simulink model "RCC_OCC_TS_TYPE1_HL"  (Simulink 7.7)
settings: Solver=ode1  StartTime=0.0  StopTime=inf  FixedStep=2e-5  RelTol=1e-3
libraries: powerlib x28, rtio_opalrt_common x4, rtlab x2
settings Model: Creator=bbkon  LastModifiedBy=USER
settings SolverCC: AutoInsertRateTranBlk=on

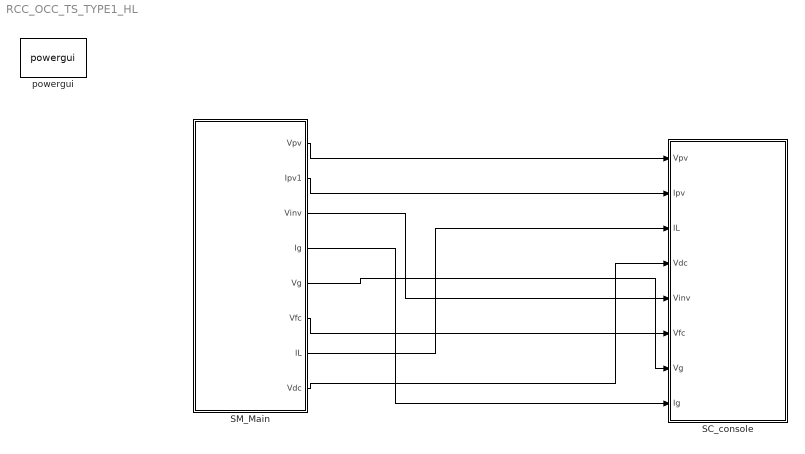
== system RCC_OCC_TS_TYPE1_HL ==
  SC_console : Subsystem
  SM_Main : Subsystem
  powergui : powerlib/powergui  Priority=1  SystemSampleTime=-1  SimulationMode=Discrete  SampleTime=2e-5  frequency=60  SPID=off  DisableSnubberDevices=off  DisableRonSwitches=off  DisableVfSwitches=off  SwTol=0  Interpol=off  DisplayEquations=off  FunctionMessages=off  frequencyindice=0  Pbase=100e6  ErrMax=1e-4  Iterations=50  UnitsV=kV  UnitsW=MW  echomessages=off  HookPort=off  EnableUseOfTLC=off  x0status=blocks  RestoreLinks=warning  ResistiveCurrentMeasurement=off  Ylog=off  Xlog=on  ShowGrid=off  save=off  variable=ZData  ZoomFFT=off  StartTime=0.0  cycles=1  DisplayStyle=1  FreqAxis=off  MaxFrequency=1000  frequencyindicesteady=1  display=off  methode=off
  wires:
  SM_Main/1(Vpv) -> SC_console/1(Vpv)
  SM_Main/2(Ipv1) -> SC_console/2(Ipv)
  SM_Main/3(Vinv) -> SC_console/5(Vinv)
  SM_Main/4(Ig) -> SC_console/8(Ig)
  SM_Main/5(Vg) -> SC_console/7(Vg)
  SM_Main/6(Vfc) -> SC_console/6(Vfc)
  SM_Main/7(IL) -> SC_console/3(IL)
  SM_Main/8(Vdc) -> SC_console/4(Vdc)

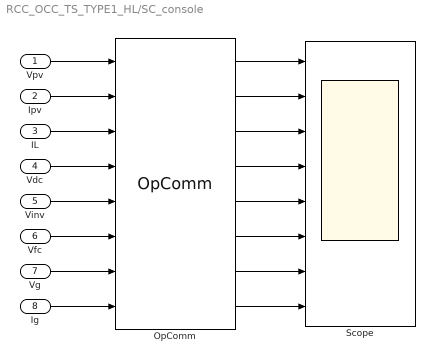
== system RCC_OCC_TS_TYPE1_HL/SC_console ==
  Vpv : Inport
  Ipv : Inport  Port=2
  IL : Inport  Port=3
  Vdc : Inport  Port=4
  Vinv : Inport  Port=5
  Vfc : Inport  Port=6
  Vg : Inport  Port=7
  Ig : Inport  Port=8
  OpComm : rtlab/OpComm  SystemSampleTime=-1  nbport=8  groupe_acq=1  subsys_rate=0  st=0  Synchronization=on  Interpolation=on  Threshold=1.0  Missed_Data=off  Sim_Time=off  Samples=off  dynSigOut=off  from_console=0  warning_done=off  writeOpCommFile=off  Offset=off
  Scope : Scope  NumInputPorts=8
      settings: YMin=80~7.25~6.5~394~-500~399~-400~-7.5  YMax=125~9.75~11.5~405~500~408~400~7.5
  wires:
  Vpv/1 -> OpComm/1
  Ipv/1 -> OpComm/2
  IL/1 -> OpComm/3
  Vdc/1 -> OpComm/4
  Vinv/1 -> OpComm/5
  Vfc/1 -> OpComm/6
  Vg/1 -> OpComm/7
  Ig/1 -> OpComm/8
  OpComm/1 -> Scope/1
  OpComm/2 -> Scope/2
  OpComm/3 -> Scope/3
  OpComm/4 -> Scope/4
  OpComm/5 -> Scope/5
  OpComm/6 -> Scope/6
  OpComm/7 -> Scope/7
  OpComm/8 -> Scope/8

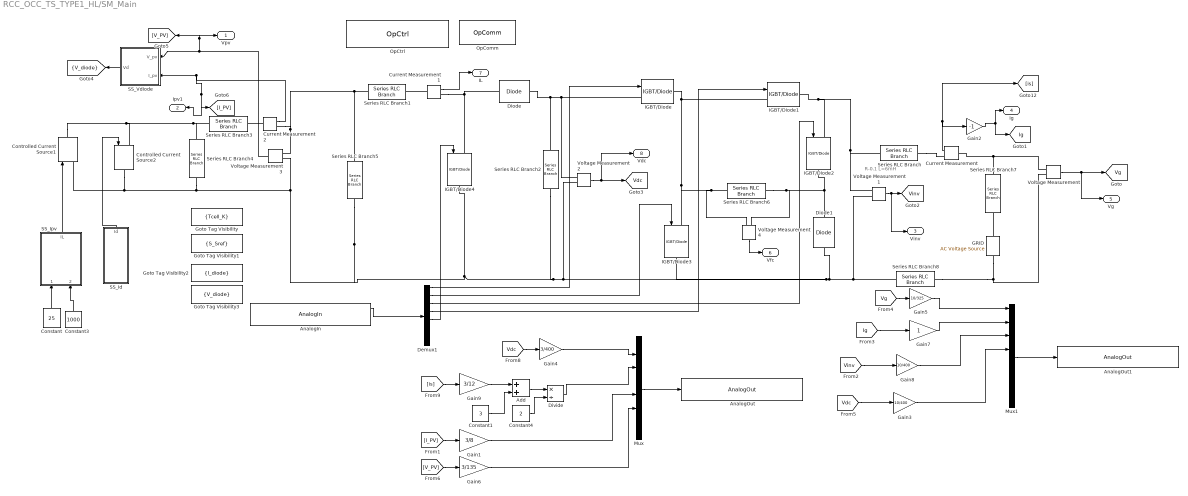
== system RCC_OCC_TS_TYPE1_HL/SM_Main ==
  note: R-0.1 L=6mH
  Add : Sum
  AnalogIn : rtio_opalrt_common/AnalogIn  CtrlName='OpCtrl'  portNb=1  FcnNos=Slot 2 Module A Subsection 1  size=16  maxcount=8  count=8  numchan=8  sampleTime=2e-5
      settings: AttributesFormatString=%<CtrlName>
  AnalogOut : rtio_opalrt_common/AnalogOut  CtrlName='OpCtrl'  portNb=1  FcnNos=Slot 2 Module B Subsection 1  size=16  maxcount=8  count=8  numchan=8  israngeinput=off  voltagerange=[-16 ... 16]  slot=1  side=1  mismatch=0  slotside=Slot_2_Module_B
      settings: AttributesFormatString=%<CtrlName>
  AnalogOut1 : rtio_opalrt_common/AnalogOut  CtrlName='OpCtrl'  portNb=2  FcnNos=Slot 2 Module B Subsection 2  size=16  maxcount=8  count=8  numchan=8  israngeinput=off  voltagerange=[-16 ... 16]  slot=1  side=1  mismatch=0  slotside=Slot_2_Module_B
      settings: AttributesFormatString=%<CtrlName>
  Constant : Constant  Value=25
  Constant1 : Constant  Value=3  SampleTime=-1
  Constant3 : Constant  Value=1000
  Constant4 : Constant  Value=2  SampleTime=-1
  Controlled Current Source1 : powerlib/Electrical Sources/Controlled Current Source  SystemSampleTime=-1  Initialize=on  Source_Type=AC  Amplitude=0  Phase=0  Frequency=0  Measurements=None
  Controlled Current Source2 : powerlib/Electrical Sources/Controlled Current Source  SystemSampleTime=-1  Initialize=on  Source_Type=AC  Amplitude=0  Phase=0  Frequency=0  Measurements=None
  Current Measurement : powerlib/Measurements/Current Measurement  SystemSampleTime=-1  PhasorSimulation=off  OutputType=Complex  PSBequivalent=0
  Current Measurement1 : powerlib/Measurements/Current Measurement  SystemSampleTime=-1  PhasorSimulation=off  OutputType=Complex  PSBequivalent=0
  Current Measurement2 : powerlib/Measurements/Current Measurement  SystemSampleTime=-1  PhasorSimulation=off  OutputType=Complex  PSBequivalent=0
  Demux1 : Demux  Outputs=8
  Diode : powerlib/Power Electronics/Diode  SystemSampleTime=-1  Ron=0.001  Lon=0  Vf=0.8  IC=0  UseSnubber=off  Rs=500  Cs=250e-9  Measurements=off
  Diode1 : powerlib/Power Electronics/Diode  SystemSampleTime=-1  Ron=0.001  Lon=0  Vf=0.8  IC=0  UseSnubber=off  Rs=500  Cs=250e-9  Measurements=off
  Divide : Product  Inputs=*/
  GRID : powerlib/Electrical Sources/AC Voltage Source  SystemSampleTime=-1  Amplitude=325  Phase=0  Frequency=50  SampleTime=0  Measurements=None
  Gain1 : Gain  Gain=3/8
  Gain2 : Gain  Gain=-1
  Gain3 : Gain  Gain=10/400
  Gain4 : Gain  Gain=3/400
  Gain5 : Gain  Gain=10/325
  Gain6 : Gain  Gain=3/135
  Gain7 : Gain
  Gain8 : Gain  Gain=10/400
  Gain9 : Gain  Gain=3/12
  Goto Tag Visibility : GotoTagVisibility  GotoTag=Tcell_K
  Goto Tag Visibility1 : GotoTagVisibility  GotoTag=S_Sref
  Goto Tag Visibility2 : GotoTagVisibility  GotoTag=I_diode
  Goto Tag Visibility3 : GotoTagVisibility  GotoTag=V_diode
  IGBT/Diode{,1..4} (5 alike) : powerlib/Power Electronics/IGBT//Diode  SystemSampleTime=-1  Ron=1e-3  Rs=1e5  Cs=inf  Measurements=off
  Mux : Mux  Inputs=8
  Mux1 : Mux  Inputs=8
  OpComm : rtlab/OpComm  SystemSampleTime=-1  nbport=0  groupe_acq=1  subsys_rate=0  st=0  Synchronization=on  Interpolation=on  Threshold=1.0  Missed_Data=off  Sim_Time=off  Samples=off  dynSigOut=off  from_console=0  warning_done=off  writeOpCommFile=off  Offset=off
  OpCtrl : rtio_opalrt_common/OpCtrl  CtrlName='OpCtrl'  boardid=0  BitstreamFilename=MMPK7_1-EX-0001-2_2_2_15-SERIES100-100-09.bin  numconfig=-1  mode=Master  externalClock=off  decimRtsi=0  calibIO=off  SampleTime=0  loadinport=-1  BoardType=OP4500  SecondaryPresent=off  sync_type=Audio
  SS_Id : Subsystem
  SS_Ipv : Subsystem
  SS_Vdiode : Subsystem
  Series RLC Branch : powerlib/Elements/Series RLC Branch  PhysicalDomain=powersysdomain  SubClassName=unknown  LeftPortType=p1  RightPortType=p1  LConnTagsString=__new0  RConnTagsString=__new0  BranchType=RL  Resistance=0.1  Inductance=3.825e-3  SetiL0=off  InitialCurrent=0  Capacitance=1e-6  Setx0=off  InitialVoltage=0  Measurements=None
  Series RLC Branch1 : powerlib/Elements/Series RLC Branch  PhysicalDomain=powersysdomain  SubClassName=unknown  LeftPortType=p1  RightPortType=p1  LConnTagsString=__new0  RConnTagsString=__new0  BranchType=RL  Resistance=0.1  Inductance=5.81e-3  SetiL0=off  InitialCurrent=0  Capacitance=1e-6  Setx0=off  InitialVoltage=0  Measurements=None
  Series RLC Branch2 : powerlib/Elements/Series RLC Branch  PhysicalDomain=powersysdomain  SubClassName=unknown  LeftPortType=p1  RightPortType=p1  LConnTagsString=__new0  RConnTagsString=__new0  BranchType=RC  Resistance=0.0001  Inductance=6e-3  SetiL0=off  InitialCurrent=0  Capacitance=500e-6  Setx0=off  InitialVoltage=0  Measurements=None
  Series RLC Branch3 : powerlib/Elements/Series RLC Branch  PhysicalDomain=powersysdomain  SubClassName=unknown  LeftPortType=p1  RightPortType=p1  LConnTagsString=__new0  RConnTagsString=__new0  BranchType=R  Resistance=1.7242  Inductance=1e-3  SetiL0=off  InitialCurrent=0  Capacitance=1e-6  Setx0=off  InitialVoltage=0  Measurements=None
  Series RLC Branch4 : powerlib/Elements/Series RLC Branch  PhysicalDomain=powersysdomain  SubClassName=unknown  LeftPortType=p1  RightPortType=p1  LConnTagsString=__new0  RConnTagsString=__new0  BranchType=R  Resistance=15068  Inductance=1e-3  SetiL0=off  InitialCurrent=0  Capacitance=1e-6  Setx0=off  InitialVoltage=0  Measurements=None
  Series RLC Branch5 : powerlib/Elements/Series RLC Branch  PhysicalDomain=powersysdomain  SubClassName=unknown  LeftPortType=p1  RightPortType=p1  LConnTagsString=__new0  RConnTagsString=__new0  BranchType=RC  Resistance=0.0001  Inductance=7.5e-3  SetiL0=off  InitialCurrent=0  Capacitance=15e-6  Setx0=off  InitialVoltage=0  Measurements=None
  Series RLC Branch6 : powerlib/Elements/Series RLC Branch  PhysicalDomain=powersysdomain  SubClassName=unknown  LeftPortType=p1  RightPortType=p1  LConnTagsString=__new0  RConnTagsString=__new0  BranchType=C  Resistance=0.1  Inductance=6e-3  SetiL0=off  InitialCurrent=0  Capacitance=1100e-6  Setx0=off  InitialVoltage=0  Measurements=None
  Series RLC Branch7 : powerlib/Elements/Series RLC Branch  PhysicalDomain=powersysdomain  SubClassName=unknown  LeftPortType=p1  RightPortType=p1  LConnTagsString=__new0  RConnTagsString=__new0  BranchType=R  Resistance=0.01  Inductance=25e-3  SetiL0=off  InitialCurrent=0  Capacitance=1e-6  Setx0=off  InitialVoltage=0  Measurements=None
  Series RLC Branch8 : powerlib/Elements/Series RLC Branch  PhysicalDomain=powersysdomain  SubClassName=unknown  LeftPortType=p1  RightPortType=p1  LConnTagsString=__new0  RConnTagsString=__new0  BranchType=RL  Resistance=0.1  Inductance=3.825e-3  SetiL0=off  InitialCurrent=0  Capacitance=1e-6  Setx0=off  InitialVoltage=0  Measurements=None
  Voltage Measurement{,1..4} (5 alike) : powerlib/Measurements/Voltage Measurement  SystemSampleTime=-1  PhasorSimulation=off  OutputType=Complex  PSBequivalent=0
  Vpv : Outport
  Ipv1 : Outport  Port=2
  Vinv : Outport  Port=3
  Ig : Outport  Port=4
  Vg : Outport  Port=5
  Vfc : Outport  Port=6
  IL : Outport  Port=7
  Vdc : Outport  Port=8
  tag scope: Ig=global, V_diode=scoped, Vdc=global, Vg=global, Vinv=global
  wires:
  Voltage Measurement/1 -> Vg/1, [Vg]
  Voltage Measurement1/1 -> [Vinv], Vinv/1
  Voltage Measurement2/1 -> Vdc/1, [Vdc]
  Voltage Measurement3/1 -> SS_Vdiode/1(V_pv), [V_PV], Vpv/1
  SS_Ipv/1(IL) -> Controlled Current Source1/1
  SS_Id/1(Id) -> Controlled Current Source2/1
  SS_Vdiode/1(Vd) -> [V_diode]
  Current Measurement2/1 -> SS_Vdiode/2(I_pv), [I_PV], Ipv1/1
  Current Measurement1/1 -> IL/1
  Demux1/3 -> IGBT/Diode2/1
  Constant/1 -> SS_Ipv/1(Temperature)
  Voltage Measurement4/1 -> Vfc/1
  Current Measurement/1 -> [is], Gain2/1
  Gain2/1 -> [Ig], Ig/1
  AnalogIn/1 -> Demux1/1
  Demux1/1 -> IGBT/Diode/1
  Demux1/2 -> IGBT/Diode3/1
  Demux1/4 -> IGBT/Diode1/1
  Demux1/5 -> IGBT/Diode4/1
  [Vinv] -> Gain8/1
  [Ig] -> Gain7/1
  Mux1/1 -> AnalogOut1/1
  Gain5/1 -> Mux1/1
  Gain7/1 -> Mux1/2
  Gain8/1 -> Mux1/3
  [Vg] -> Gain5/1
  [Vdc] -> Gain3/1
  Gain3/1 -> Mux1/4
  Mux/1 -> AnalogOut/1
  [Vdc] -> Gain4/1
  [is] -> Gain9/1
  Gain9/1 -> Add/1
  Constant1/1 -> Add/2
  Add/1 -> Divide/1
  Constant4/1 -> Divide/2
  Gain4/1 -> Mux/2
  Divide/1 -> Mux/3
  [I_PV] -> Gain1/1
  Gain1/1 -> Mux/5
  [V_PV] -> Gain6/1
  Gain6/1 -> Mux/6
  Constant3/1 -> SS_Ipv/2(Irradiance)
  connections:
  Series RLC Branch8/RConn1 -- GRID/LConn1 -- Voltage Measurement/LConn2
  Controlled Current Source1/RConn1 -- Series RLC Branch4/LConn1 -- Series RLC Branch3/LConn1 -- Controlled Current Source2/LConn1
  Series RLC Branch/RConn1 -- Current Measurement/RConn1
  Voltage Measurement/LConn1 -- Current Measurement/LConn1 -- Series RLC Branch7/LConn1
  Current Measurement1/LConn1 -- Series RLC Branch1/RConn1
  Current Measurement1/RConn1 -- Diode/LConn1 -- IGBT/Diode4/LConn1
  Current Measurement2/LConn1 -- Series RLC Branch3/RConn1
  Current Measurement2/RConn1 -- Series RLC Branch5/LConn1 -- Series RLC Branch1/LConn1 -- Voltage Measurement3/LConn1
  Diode/RConn1 -- Voltage Measurement2/LConn1 -- IGBT/Diode/LConn1 -- Series RLC Branch2/LConn1
  Diode1/LConn1 -- IGBT/Diode2/RConn1 -- Series RLC Branch6/RConn1 -- Voltage Measurement4/LConn2
  IGBT/Diode/RConn1 -- IGBT/Diode3/LConn1 -- Series RLC Branch6/LConn1 -- Voltage Measurement4/LConn1 -- IGBT/Diode1/LConn1
  IGBT/Diode1/RConn1 -- Series RLC Branch/LConn1 -- Voltage Measurement1/LConn1 -- IGBT/Diode2/LConn1
  Voltage Measurement1/LConn2 -- Controlled Current Source1/LConn1 -- Controlled Current Source2/RConn1 -- Series RLC Branch4/RConn1 -- Voltage Measurement3/LConn2 -- Series RLC Branch5/RConn1 -- IGBT/Diode4/RConn1 -- Series RLC Branch2/RConn1 -- Voltage Measurement2/LConn2 -- IGBT/Diode3/RConn1 -- Diode1/RConn1 -- Series RLC Branch8/LConn1
  GRID/RConn1 -- Series RLC Branch7/RConn1

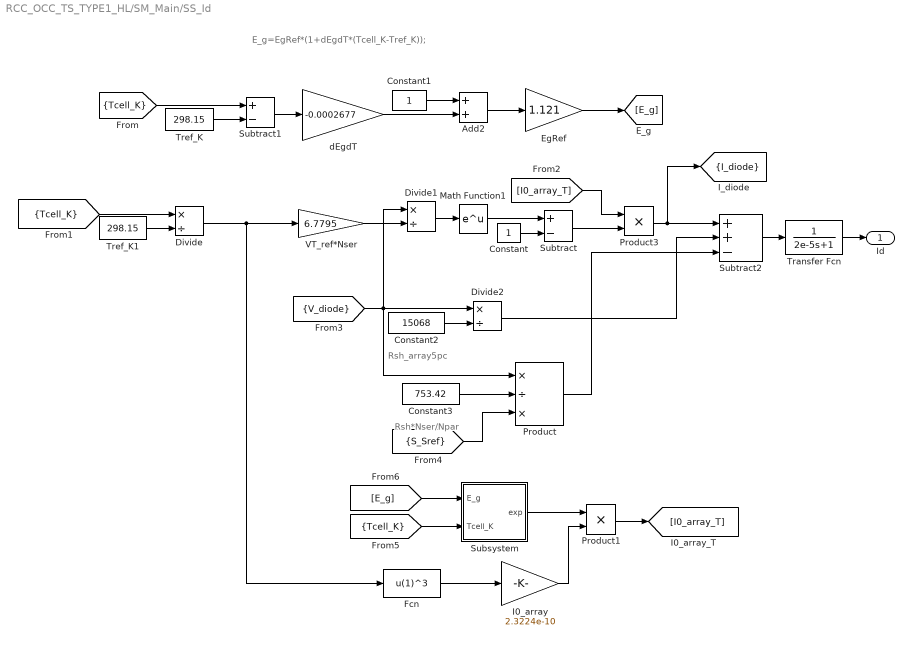
== system RCC_OCC_TS_TYPE1_HL/SM_Main/SS_Id ==
  note: E_g=EgRef*(1+dEgdT*(Tcell_K-Tref_K));
  note: Rsh_array5pc
  note: Rsh*Nser/Npar
  Add2 : Sum
  Constant : Constant
  Constant1 : Constant
  Constant2 : Constant  Value=15068
  Constant3 : Constant  Value=753.42
  Divide : Product  Inputs=*/
  Divide1 : Product  Inputs=*/
  Divide2 : Product  Inputs=*/
  EgRef : Gain  Gain=1.121
  Fcn : Fcn  Expr=u(1)^3
  I0_array : Gain  Gain=2.3224e-10
  Math Function1 : Math  SaturateOnIntegerOverflow=on
  Product : Product  Inputs=*/*  RndMeth=Zero
  Product1 : Product  RndMeth=Zero
  Product3 : Product  RndMeth=Zero
  Subsystem : Subsystem
  Subtract : Sum  Inputs=+-
  Subtract1 : Sum  Inputs=+-
  Subtract2 : Sum  Inputs=++-
  Transfer Fcn : TransferFcn  Denominator=[2e-5, 1]
  Tref_K : Constant  Value=298.15
  Tref_K1 : Constant  Value=298.15
  VT_ref*Nser : Gain  Gain=6.7795
  dEgdT : Gain  Gain=-0.0002677
  Id : Outport
  tag scope: I_diode=scoped
  wires:
  Constant/1 -> Subtract/2
  [Tcell_K] -> Subtract1/1
  Tref_K/1 -> Subtract1/2
  Subtract1/1 -> dEgdT/1
  dEgdT/1 -> Add2/2
  Constant1/1 -> Add2/1
  Add2/1 -> EgRef/1
  EgRef/1 -> [E_g]
  Tref_K1/1 -> Divide/2
  [Tcell_K] -> Divide/1
  Divide/1 -> VT_ref*Nser/1, Fcn/1
  VT_ref*Nser/1 -> Divide1/2
  Divide1/1 -> Math Function1/1
  Math Function1/1 -> Subtract/1
  Subtract2/1 -> Transfer Fcn/1
  Transfer Fcn/1 -> Id/1
  Product/1 -> Subtract2/3
  Product3/1 -> Subtract2/1, [I_diode]
  Subtract/1 -> Product3/2
  [I0_array_T] -> Product3/1
  [V_diode] -> Product/1, Divide1/1, Divide2/1
  Divide2/1 -> Subtract2/2
  Constant2/1 -> Divide2/2
  Constant3/1 -> Product/2
  [S_Sref] -> Product/3
  [E_g] -> Subsystem/1(E_g)
  [Tcell_K] -> Subsystem/2(Tcell_K)
  Subsystem/1(exp) -> Product1/1
  Fcn/1 -> I0_array/1
  I0_array/1 -> Product1/2
  Product1/1 -> [I0_array_T]

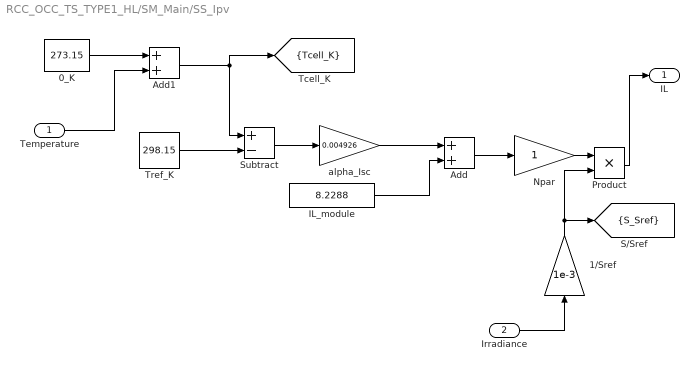
== system RCC_OCC_TS_TYPE1_HL/SM_Main/SS_Ipv ==
  Temperature : Inport
  Irradiance : Inport  Port=2
  0_K : Constant  Value=273.15
  1/Sref : Gain  Gain=1e-3
  Add : Sum
  Add1 : Sum
  IL_module : Constant  Value=8.2288
  Npar : Gain
  Product : Product  RndMeth=Zero
  Subtract : Sum  Inputs=+-
  Tref_K : Constant  Value=298.15
  alpha_Isc : Gain  Gain=0.004926
  IL : Outport
  tag scope: S_Sref=scoped, Tcell_K=scoped
  wires:
  Temperature/1 -> Add1/2
  Subtract/1 -> alpha_Isc/1
  IL_module/1 -> Add/2
  0_K/1 -> Add1/1
  Add1/1 -> Subtract/1, [Tcell_K]
  Tref_K/1 -> Subtract/2
  alpha_Isc/1 -> Add/1
  Add/1 -> Npar/1
  Npar/1 -> Product/1
  Irradiance/1 -> 1/Sref/1
  1/Sref/1 -> Product/2, [S_Sref]
  Product/1 -> IL/1

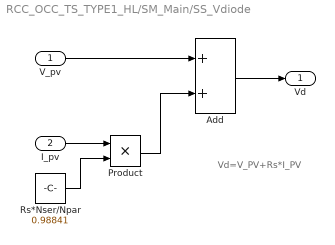
== system RCC_OCC_TS_TYPE1_HL/SM_Main/SS_Vdiode ==
  note: Vd=V_PV+Rs*I_PV
  V_pv : Inport
  I_pv : Inport  Port=2
  Add : Sum
  Product : Product  RndMeth=Zero
  Rs*Nser/Npar : Constant  Value=0.98841
  Vd : Outport
  wires:
  I_pv/1 -> Product/1
  Rs*Nser/Npar/1 -> Product/2
  Product/1 -> Add/2
  V_pv/1 -> Add/1
  Add/1 -> Vd/1

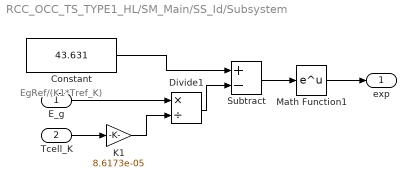
== system RCC_OCC_TS_TYPE1_HL/SM_Main/SS_Id/Subsystem ==
  note: EgRef/(K1*Tref_K)
  E_g : Inport
  Tcell_K : Inport  Port=2
  Constant : Constant  Value=43.631
  Divide1 : Product  Inputs=*/
  K1 : Gain  Gain=8.6173e-05
  Math Function1 : Math  SaturateOnIntegerOverflow=on
  Subtract : Sum  Inputs=+-
  exp : Outport
  wires:
  E_g/1 -> Divide1/1
  Tcell_K/1 -> K1/1
  K1/1 -> Divide1/2
  Divide1/1 -> Subtract/2
  Constant/1 -> Subtract/1
  Subtract/1 -> Math Function1/1
  Math Function1/1 -> exp/1
